simulink model "gtm_design"  (R2021b)
settings: Solver=VariableStepAuto  StartTime=0.0  StopTime=10.0  MinStep=0.00999  RelTol=1e-3
StopFcn:
  | MWSout=grabmws(bdroot);
  | MWSout.lastrun=datestr(now);
values from neighbouring files (symbols this model uses):
  knots2fps = 1.68781    [setup.m]
  s = tf('s')    [setup.m]
undefined symbols (not defined in the file or in its folder): Aero, aftfuel, aftfuel_pos, AILL, AILLC, AILR, AILRC, alpha_deg, alt0, altitude_ft, Ax_g, Ay_g, Az_g, b, beta_deg, bias, BRAKEC, Cbar, cg_pos0, cg_shift_gear, ControlMode, DamageCase, DamageModels, DamageOnsetTime, deltc, Earth, ELLIB, ELLIBC, ELLOB, ELLOBC, ELRIB, ELRIBC, ELROB, ELROBC, engl_ang, engl_pos, engr_ang, engr_pos, etas0, etas1, etasc_feedthrough, FLAPLC, FLAPLIB, FLAPLOB, FLAPRC, FLAPRIB, FLAPROB, FlightMode, FuelUsed_Init, fwdfuel, fwdfuel_pos, GEAR, GEARC, Inertia0, Inertia_shift_gear, Ixx_model, Iyy_model, Izz_model, KTAS, LandingGear ... (+66)
libraries: simulink_extras x98, LPVBlockLibrary x54, simulink_need_slupdate x30, aerolibconvert2 x27, simulink x7, aerolibtransform2 x6, uavalgslib x4, UserContent_lib x2, robotcorelib x1, uavutilslib x1
(part 7 of 9)

== system gtm_design/Guidance/Autopilot Trajectory Tracking/Orbit Following/Pose ==
  Feedback : Inport
  Bus Creator : BusCreator  Inputs=8
  Bus Selector : BusSelector  OutputSignals=AirData.KTAS
  Bus Selector1 : BusSelector  OutputSignals=MIDG.NAV_Vu_mps,MIDG.NAV_Vn_mps,MIDG.NAV_Ve_mps
  Bus Selector2 : BusSelector  OutputSignals=MIDG.NAV_Ve_mps,MIDG.NAV_Vn_mps
  Bus Selector3 : BusSelector  OutputSignals=MIDG.NAV_latitude_deg,MIDG.NAV_longitude_deg,MIDG.NAV_altitude_m
  Bus Selector4 : BusSelector  OutputSignals=MIDG.phi_deg,MAG3.p_deg
  Bus Selector6 : BusSelector  OutputSignals=North,East,Height,HeadingAngle  OutputAsBus=on
  Bus to Vector : BusToVector
  Bus to Vector1 : BusToVector
  Bus to Vector2 : BusToVector
  Constant1 : Constant  Value=[37.827926944;-75.494061666]
  Constant2 : Constant  Value=0
  Constant3 : Constant  Value=0
  Degrees to Radians{,1..3} (4 alike) : simulink_extras/Transformations/Degrees to Radians
  Demux1 : Demux  Outputs=3
      settings: DisplayOption=none
  Gain : Gain  Gain=-1
  LLA to Flat Earth : aerolibtransform2/LLA to Flat Earth  units=Metric (MKS)  ptype=Earth (WGS84)  F=1/298.257223563  R=6378137  refPosPort=on  LL0=[0 10]  psi=0
      settings: SourceProductBaseCode=AE
  Map 0_1 : Subsystem
  Mux : Mux  Inputs=2
  Mux2 : Mux  Inputs=2
  Trigonometric Function1 : Trigonometry  Operator=atan2
  Trigonometric Function3 : Trigonometry  Operator=atan2
  VecNorm : Subsystem
  Velocity Conversion : aerolibconvert2/Velocity Conversion  IU=kts  OU=m/s
  fpstoknots2 : Gain  Gain=180/pi
  Pose : Outport
  wires:
  Bus Selector2/2 -> Trigonometric Function3/2  "<NAV_Vn_mps>"
  Trigonometric Function3/1 -> Map 0_1/1(I)  "gndtrack"
  Map 0_1/1(O) -> Degrees to Radians/1  "HeadingAngle"
  Bus Selector2/1 -> Trigonometric Function3/1  "<NAV_Ve_mps>"
  Feedback/1 -> Bus Selector/1, Bus Selector4/1, Bus Selector1/1, Bus Selector2/1, Bus Selector3/1
  Mux2/1 -> LLA to Flat Earth/1
  LLA to Flat Earth/1 -> Demux1/1
  Constant1/1 -> LLA to Flat Earth/4
  Bus Selector3/2 -> Mux2/2  "<NAV_longitude_deg>"
  Bus Selector3/1 -> Mux2/1  "<NAV_latitude_deg>"
  Constant3/1 -> LLA to Flat Earth/3
  Bus Selector3/3 -> LLA to Flat Earth/2  "<NAV_altitude_m>"
  Demux1/3 -> Gain/1  "Down"
  Constant2/1 -> LLA to Flat Earth/5
  Mux/1 -> VecNorm/1(I)
  VecNorm/1(O) -> Trigonometric Function1/2
  Trigonometric Function1/1 -> fpstoknots2/1  "gamma"
  Bus Selector1/3 -> Mux/2  "<NAV_Ve_mps>"
  Bus Selector1/2 -> Mux/1  "<NAV_Vn_mps>"
  Bus Selector1/1 -> Trigonometric Function1/1  "<NAV_Vu_mps>"
  Gain/1 -> Bus Creator/3  "Height"
  Demux1/2 -> Bus Creator/2  "East"
  Demux1/1 -> Bus Creator/1  "North"
  Bus Selector/1 -> Bus to Vector/1  "<KTAS>"
  fpstoknots2/1 -> Degrees to Radians1/1  "FlightPathAngle"
  Bus Selector4/2 -> Bus to Vector2/1  "<p_deg>"
  Bus Selector4/1 -> Bus to Vector1/1  "<phi_deg>"
  Bus to Vector/1 -> Velocity Conversion/1  "KTAS"
  Bus to Vector1/1 -> Degrees to Radians2/1  "RollAngle"
  Bus to Vector2/1 -> Degrees to Radians3/1  "RollAngleRate"
  Velocity Conversion/1 -> Bus Creator/4  "AirSpeed"
  Bus Selector6/1 -> Pose/1
  Bus Creator/1 -> Bus Selector6/1
  Degrees to Radians/1 -> Bus Creator/5  "HeadingAngle"
  Degrees to Radians1/1 -> Bus Creator/6  "FlightPathAngle"
  Degrees to Radians2/1 -> Bus Creator/7  "RollAngle"
  Degrees to Radians3/1 -> Bus Creator/8  "RollAngleRate"

== system gtm_design/Guidance/Autopilot Trajectory Tracking/Waypoint Following/Pose ==
  Feedback : Inport
  Bus Creator : BusCreator  Inputs=8
  Bus Selector : BusSelector  OutputSignals=AirData.KTAS
  Bus Selector1 : BusSelector  OutputSignals=MIDG.NAV_Vu_mps,MIDG.NAV_Vn_mps,MIDG.NAV_Ve_mps
  Bus Selector2 : BusSelector  OutputSignals=MIDG.NAV_Ve_mps,MIDG.NAV_Vn_mps
  Bus Selector3 : BusSelector  OutputSignals=MIDG.NAV_latitude_deg,MIDG.NAV_longitude_deg,MIDG.NAV_altitude_m
  Bus Selector4 : BusSelector  OutputSignals=MIDG.phi_deg,MAG3.p_deg
  Bus Selector6 : BusSelector  OutputSignals=North,East,Height,HeadingAngle  OutputAsBus=on
  Bus to Vector : BusToVector
  Bus to Vector1 : BusToVector
  Bus to Vector2 : BusToVector
  Constant1 : Constant  Value=[37.827926944;-75.494061666]
  Constant2 : Constant  Value=0
  Constant3 : Constant  Value=0
  Degrees to Radians{,1..3} (4 alike) : simulink_extras/Transformations/Degrees to Radians
  Demux1 : Demux  Outputs=3
      settings: DisplayOption=none
  Gain : Gain  Gain=-1
  LLA to Flat Earth : aerolibtransform2/LLA to Flat Earth  units=Metric (MKS)  ptype=Earth (WGS84)  F=1/298.257223563  R=6378137  refPosPort=on  LL0=[0 10]  psi=0
      settings: SourceProductBaseCode=AE
  Map 0_1 : Subsystem
  Mux : Mux  Inputs=2
  Mux2 : Mux  Inputs=2
  Trigonometric Function1 : Trigonometry  Operator=atan2
  Trigonometric Function3 : Trigonometry  Operator=atan2
  VecNorm : Subsystem
  Velocity Conversion : aerolibconvert2/Velocity Conversion  IU=kts  OU=m/s
  fpstoknots2 : Gain  Gain=180/pi
  Pose : Outport
  wires:
  Degrees to Radians3/1 -> Bus Creator/8  "RollAngleRate"
  Degrees to Radians2/1 -> Bus Creator/7  "RollAngle"
  Degrees to Radians1/1 -> Bus Creator/6  "FlightPathAngle"
  Degrees to Radians/1 -> Bus Creator/5  "HeadingAngle"
  Bus Creator/1 -> Bus Selector6/1
  Bus Selector6/1 -> Pose/1
  Velocity Conversion/1 -> Bus Creator/4  "AirSpeed"
  Bus to Vector2/1 -> Degrees to Radians3/1  "RollAngleRate"
  Bus to Vector1/1 -> Degrees to Radians2/1  "RollAngle"
  Bus to Vector/1 -> Velocity Conversion/1  "KTAS"
  Bus Selector4/1 -> Bus to Vector1/1  "<phi_deg>"
  Bus Selector4/2 -> Bus to Vector2/1  "<p_deg>"
  fpstoknots2/1 -> Degrees to Radians1/1  "FlightPathAngle"
  Bus Selector/1 -> Bus to Vector/1  "<KTAS>"
  Demux1/1 -> Bus Creator/1  "North"
  Demux1/2 -> Bus Creator/2  "East"
  Gain/1 -> Bus Creator/3  "Height"
  Bus Selector1/1 -> Trigonometric Function1/1  "<NAV_Vu_mps>"
  Bus Selector1/2 -> Mux/1  "<NAV_Vn_mps>"
  Bus Selector1/3 -> Mux/2  "<NAV_Ve_mps>"
  Trigonometric Function1/1 -> fpstoknots2/1  "gamma"
  VecNorm/1(O) -> Trigonometric Function1/2
  Mux/1 -> VecNorm/1(I)
  Constant2/1 -> LLA to Flat Earth/5
  Demux1/3 -> Gain/1  "Down"
  Bus Selector3/3 -> LLA to Flat Earth/2  "<NAV_altitude_m>"
  Constant3/1 -> LLA to Flat Earth/3
  Bus Selector3/1 -> Mux2/1  "<NAV_latitude_deg>"
  Bus Selector3/2 -> Mux2/2  "<NAV_longitude_deg>"
  Constant1/1 -> LLA to Flat Earth/4
  LLA to Flat Earth/1 -> Demux1/1
  Mux2/1 -> LLA to Flat Earth/1
  Feedback/1 -> Bus Selector3/1, Bus Selector2/1, Bus Selector1/1, Bus Selector4/1, Bus Selector/1
  Bus Selector2/1 -> Trigonometric Function3/1  "<NAV_Ve_mps>"
  Map 0_1/1(O) -> Degrees to Radians/1  "HeadingAngle"
  Trigonometric Function3/1 -> Map 0_1/1(I)  "gndtrack"
  Bus Selector2/2 -> Trigonometric Function3/2  "<NAV_Vn_mps>"

== system gtm_design/Guidance/Heading Control/FlightState/Map 0_1 ==
  I : Inport
  Constant : Constant  Value=2*pi
  Constant1 : Constant  Value=0
  Gain : Gain  Gain=180/pi
  Sum : Sum  Inputs=|++
  ifnegadd2pi : Switch
  O : Outport
  wires:
  I/1 -> Sum/1, ifnegadd2pi/2
  Sum/1 -> Gain/1
  ifnegadd2pi/1 -> Sum/2
  Constant/1 -> ifnegadd2pi/3
  Constant1/1 -> ifnegadd2pi/1
  Gain/1 -> O/1

== system gtm_design/Guidance/Heading Control/FlightState/VecNorm ==
  I : Inport
  Math Function2 : Math  Operator=sqrt  SignedPower=on  SaturateOnIntegerOverflow=on
  Product : Product  RndMeth=Zero
  Sum of Elements : Sum  Inputs=+
  O : Outport
  wires:
  Sum of Elements/1 -> Math Function2/1
  Product/1 -> Sum of Elements/1
  I/1 -> Product/2, Product/1
  Math Function2/1 -> O/1

== system gtm_design/Guidance/Orbit Following/Subsystem1/Map 0_1 ==
  I : Inport
  Constant : Constant  Value=2*pi
  Constant1 : Constant  Value=0
  Gain : Gain  Gain=180/pi
  Sum : Sum  Inputs=|++
  ifnegadd2pi : Switch
  O : Outport
  wires:
  Gain/1 -> O/1
  Constant1/1 -> ifnegadd2pi/1
  Constant/1 -> ifnegadd2pi/3
  ifnegadd2pi/1 -> Sum/2
  Sum/1 -> Gain/1
  I/1 -> ifnegadd2pi/2, Sum/1

== system gtm_design/Guidance/Orbit Following/Subsystem1/VecNorm ==
  I : Inport
  Math Function2 : Math  Operator=sqrt  SignedPower=on  SaturateOnIntegerOverflow=on
  Product : Product  RndMeth=Zero
  Sum of Elements : Sum  Inputs=+
  O : Outport
  wires:
  Math Function2/1 -> O/1
  I/1 -> Product/1, Product/2
  Product/1 -> Sum of Elements/1
  Sum of Elements/1 -> Math Function2/1

== system gtm_design/Guidance/Waypoint Following/Subsystem1/Map 0_1 ==
  I : Inport
  Constant : Constant  Value=2*pi
  Constant1 : Constant  Value=0
  Gain : Gain  Gain=180/pi
  Sum : Sum  Inputs=|++
  ifnegadd2pi : Switch
  O : Outport
  wires:
  I/1 -> Sum/1, ifnegadd2pi/2
  Sum/1 -> Gain/1
  ifnegadd2pi/1 -> Sum/2
  Constant/1 -> ifnegadd2pi/3
  Constant1/1 -> ifnegadd2pi/1
  Gain/1 -> O/1

== system gtm_design/Guidance/Waypoint Following/Subsystem1/VecNorm ==
  I : Inport
  Math Function2 : Math  Operator=sqrt  SignedPower=on  SaturateOnIntegerOverflow=on
  Product : Product  RndMeth=Zero
  Sum of Elements : Sum  Inputs=+
  O : Outport
  wires:
  Sum of Elements/1 -> Math Function2/1
  Product/1 -> Sum of Elements/1
  I/1 -> Product/2, Product/1
  Math Function2/1 -> O/1

== system gtm_design/Control/Controller/Control Algorithm/Hinf Autopilot/Lateral-Directional Controller ==
  cmd_autopilot_lat : Inport
  feedback : Inport  Port=2
  Bus Selector : BusSelector  OutputSignals=bet_c_deg,phi_c_deg  OutputAsBus=on
  Bus to Vector : BusToVector
  Degrees to Radians : simulink_extras/Transformations/Degrees to Radians
  Degrees to Radians1 : simulink_extras/Transformations/Degrees to Radians
  Demux : Demux  Outputs=3
  Demux1 : Demux  Outputs=2
  Demux2 : Demux  Outputs=[1 2 1]
  Full State : Subsystem
  Linear Controller : LPVBlockLibrary/LPVBlock  sys=Klat4hinf  plist={'rho1_sas_param';'rho2_alt_param';'rho3_mor_param'}  x0=0
      settings: SourceProductName=LPVTools Blocks
  Mux : Mux  Inputs=2
  Mux1 : Mux  Inputs=2
  Mux2 : Mux  Inputs=2
  Scheduling Parameter : Subsystem
  Sum : Sum  Inputs=|+-
  Sum1 : Sum  Inputs=|+-
  Sum2 : Sum  Inputs=|++
  Sum3 : Sum  Inputs=|+-
  Trim Command : Subsystem
  Trim Input : Subsystem
  Trim State : Subsystem
  feedback1 : InportShadow  Port=2
  AILC : Outport
  RUDC : Outport  Port=2
  SPANAC : Outport  Port=3
  wires:
  Demux/1 -> AILC/1
  Degrees to Radians1/1 -> Mux1/2  "phi_c_rad"
  Degrees to Radians/1 -> Mux1/1  "bet_c_rad"
  feedback/1 -> Scheduling Parameter/1(feedback)
  cmd_autopilot_lat/1 -> Bus Selector/1
  Bus Selector/1 -> Bus to Vector/1  "r"
  feedback1/1 -> Full State/1(feedback)
  Full State/1(x) -> Sum1/1  "x"
  Sum1/1 -> Demux2/1  "dx"
  Demux/2 -> RUDC/1
  Demux/3 -> SPANAC/1
  Scheduling Parameter/1(rho) -> [rho]
  [rho] -> Trim Command/1(rho)
  [rho] -> Trim Input/1(rho)
  [rho] -> Trim State/1(rho)
  [rho] -> Linear Controller/2
  Sum2/1 -> Demux/1  "u"
  Trim Input/1(x_eq) -> Sum2/2
  Sum/1 -> Sum3/1  "dr"
  Mux/1 -> Linear Controller/1
  Trim State/1(x_eq) -> Sum1/2  "x_eq"
  Linear Controller/1 -> Sum2/1  "du"
  Mux1/1 -> Sum/1  "r"
  Trim Command/1(r_eq) -> Sum/2
  Bus to Vector/1 -> Demux1/1  "r"
  Demux1/1 -> Degrees to Radians/1  "bet_c_deg"
  Demux1/2 -> Degrees to Radians1/1  "phi_c_deg"
  Mux2/1 -> Sum3/2
  Sum3/1 -> Mux/1  "dx"
  Demux2/2 -> Mux/2
  Demux2/1 -> Mux2/1
  Demux2/3 -> Mux2/2

== system gtm_design/Control/Controller/Control Algorithm/Hinf Autopilot/Longitudinal Controller ==
  cmd_autopilot_lon : Inport
  feedback : Inport  Port=2
  Bus Selector : BusSelector  OutputSignals=tas_c_knot,alt_c_ft  OutputAsBus=on
  Bus to Vector : BusToVector
  Demux : Demux  Outputs=2
  Demux1 : Demux  Outputs=2
  Demux2 : Demux  Outputs=[1 3 1]
  Full State : Subsystem
  Linear Controller : LPVBlockLibrary/LPVBlock  sys=Klon5hinf  plist={'rho1_sas_param';'rho2_alt_param';'rho3_mor_param'}  x0=0
      settings: SourceProductName=LPVTools Blocks
  Mux : Mux  Inputs=2
  Mux1 : Mux  Inputs=2
  Mux2 : Mux  Inputs=2
  Scheduling Parameter : Subsystem
  Sum : Sum  Inputs=|+-
  Sum1 : Sum  Inputs=|+-
  Sum2 : Sum  Inputs=|++
  Sum3 : Sum  Inputs=|+-
  Trim Command : Subsystem
  Trim Input : Subsystem
  Trim State : Subsystem
  feedback1 : InportShadow  Port=2
  knotstofps : Gain  Gain=knots2fps
  THROTC : Outport
  ELLC : Outport  Port=2
  wires:
  Demux2/3 -> Mux2/2
  Demux2/1 -> Mux2/1
  Demux2/2 -> Mux/2
  Sum3/1 -> Mux/1  "dx"
  Mux2/1 -> Sum3/2
  knotstofps/1 -> Mux1/1  "tas_trim_fps"
  Demux1/1 -> knotstofps/1
  Bus to Vector/1 -> Demux1/1  "r"
  Trim Command/1(r_eq) -> Sum/2
  Mux1/1 -> Sum/1  "r"
  Linear Controller/1 -> Sum2/1  "du"
  Trim State/1(x_eq) -> Sum1/2  "x_eq"
  Mux/1 -> Linear Controller/1
  Sum/1 -> Sum3/1  "dr"
  Trim Input/1(u_eq) -> Sum2/2
  Sum2/1 -> Demux/1  "u"
  [rho] -> Linear Controller/2
  [rho] -> Trim State/1(rho)
  [rho] -> Trim Input/1(rho)
  [rho] -> Trim Command/1(rho)
  Scheduling Parameter/1(rho) -> [rho]
  Demux/2 -> ELLC/1
  Demux/1 -> THROTC/1
  Sum1/1 -> Demux2/1  "dx"
  Full State/1(x) -> Sum1/1  "x"
  feedback1/1 -> Full State/1(feedback)
  Bus Selector/1 -> Bus to Vector/1  "r"
  cmd_autopilot_lon/1 -> Bus Selector/1
  feedback/1 -> Scheduling Parameter/1(feedback)
  Demux1/2 -> Mux1/2

== system gtm_design/Control/Controller/Control Algorithm/Hinf CAS/Lateral-Directional Controller ==
  cmd_cas_lat : Inport
  feedback : Inport  Port=2
  Bus Selector : BusSelector  OutputSignals=bet_c_deg,p_c_deg  OutputAsBus=on
  Bus to Vector : BusToVector
  Degrees to Radians : simulink_extras/Transformations/Degrees to Radians
  Degrees to Radians1 : simulink_extras/Transformations/Degrees to Radians
  Demux : Demux  Outputs=3
  Demux1 : Demux  Outputs=2
  Demux2 : Demux  Outputs=[2 1]
  Full State : Subsystem
  Linear Controller : LPVBlockLibrary/LPVBlock  sys=Klat3hinf  plist={'rho1_sas_param';'rho2_alt_param';'rho3_mor_param'}  x0=0
      settings: SourceProductName=LPVTools Blocks
  Mux : Mux  Inputs=2
  Mux1 : Mux  Inputs=2
  Scheduling Parameter : Subsystem
  Sum : Sum  Inputs=|+-
  Sum1 : Sum  Inputs=|+-
  Sum2 : Sum  Inputs=|++
  Sum3 : Sum  Inputs=|+-
  Trim Command : Subsystem
  Trim Input : Subsystem
  Trim State : Subsystem
  feedback1 : InportShadow  Port=2
  AILC : Outport
  RUDC : Outport  Port=2
  SPANAC : Outport  Port=3
  wires:
  Sum3/1 -> Mux/1  "dx"
  Demux1/2 -> Degrees to Radians1/1  "p_c_deg"
  Demux1/1 -> Degrees to Radians/1  "bet_c_deg"
  Bus to Vector/1 -> Demux1/1  "r"
  Trim Command/1(r_eq) -> Sum/2
  Mux1/1 -> Sum/1  "r"
  Linear Controller/1 -> Sum2/1  "du"
  Trim State/1(x_eq) -> Sum1/2  "x_eq"
  Mux/1 -> Linear Controller/1
  Sum/1 -> Sum3/1  "dr"
  Trim Input/1(x_eq) -> Sum2/2
  Sum2/1 -> Demux/1  "u"
  [rho] -> Linear Controller/2
  [rho] -> Trim State/1(rho)
  [rho] -> Trim Input/1(rho)
  [rho] -> Trim Command/1(rho)
  Scheduling Parameter/1(rho) -> [rho]
  Demux/3 -> SPANAC/1
  Demux/2 -> RUDC/1
  Sum1/1 -> Demux2/1  "dx"
  Full State/1(x) -> Sum1/1  "x"
  feedback1/1 -> Full State/1(feedback)
  Bus Selector/1 -> Bus to Vector/1  "r"
  cmd_cas_lat/1 -> Bus Selector/1
  feedback/1 -> Scheduling Parameter/1(feedback)
  Degrees to Radians/1 -> Mux1/1  "bet_c_rad"
  Degrees to Radians1/1 -> Mux1/2  "p_c_rad"
  Demux/1 -> AILC/1
  Demux2/2 -> Mux/2
  Demux2/1 -> Sum3/2

== system gtm_design/Control/Controller/Control Algorithm/Hinf CAS/Longitudinal Controller ==
  cmd_cas_lon : Inport
  feedback : Inport  Port=2
  Bus Selector : BusSelector  OutputSignals=an_c_g  OutputAsBus=on
  Bus to Vector : BusToVector
  Constant : Constant  Value=deltc
  Demux2 : Demux  Outputs=[2 1]
  Full State : Subsystem
  Gain : Gain  Gain=-1
  Linear Controller : LPVBlockLibrary/LPVBlock  sys=Klon2hinf  plist={'rho1_sas_param';'rho2_alt_param';'rho3_mor_param'}  x0=0
      settings: SourceProductName=LPVTools Blocks
  Mux : Mux  Inputs=2
  Scheduling Parameter : Subsystem
  Sum : Sum  Inputs=|+-
  Sum1 : Sum  Inputs=|+-
  Sum2 : Sum  Inputs=|++
  Sum3 : Sum  Inputs=|+-
  Trim Command : Subsystem
  Trim Input : Subsystem
  Trim State : Subsystem
  feedback1 : InportShadow  Port=2
  knotstofps : Gain  Gain=32.174
  THROTC : Outport
  ELLC : Outport  Port=2
  wires:
  feedback/1 -> Scheduling Parameter/1(feedback)
  cmd_cas_lon/1 -> Bus Selector/1
  Bus Selector/1 -> Bus to Vector/1  "r"
  feedback1/1 -> Full State/1(feedback)
  Full State/1(y) -> Sum1/1  "y"
  Sum1/1 -> Demux2/1  "dy"
  Constant/1 -> THROTC/1
  Scheduling Parameter/1(rho) -> [rho]
  [rho] -> Trim Command/1(rho)
  [rho] -> Trim Input/1(rho)
  [rho] -> Trim State/1(rho)
  [rho] -> Linear Controller/2
  Sum2/1 -> ELLC/1  "u"
  Trim Input/1(u_eq) -> Sum2/2
  Sum/1 -> Sum3/1  "dr"
  Mux/1 -> Linear Controller/1
  Trim State/1(x_eq) -> Sum1/2  "x_eq"
  Linear Controller/1 -> Sum2/1  "du"
  knotstofps/1 -> Sum/1  "r"
  Trim Command/1(r_eq) -> Sum/2  "r_eq"
  Bus to Vector/1 -> knotstofps/1  "an_c_g"
  Sum3/1 -> Mux/1  "dx"
  Demux2/2 -> Gain/1
  Demux2/1 -> Mux/2
  Gain/1 -> Sum3/2

== system gtm_design/Control/Controller/Control Algorithm/LPV Autopilot/Lateral-Directional Controller ==
  cmd_autopilot_lat : Inport
  feedback : Inport  Port=2
  Bus Selector : BusSelector  OutputSignals=bet_c_deg,phi_c_deg  OutputAsBus=on
  Bus to Vector : BusToVector
  Degrees to Radians : simulink_extras/Transformations/Degrees to Radians
  Degrees to Radians1 : simulink_extras/Transformations/Degrees to Radians
  Demux : Demux  Outputs=3
  Demux1 : Demux  Outputs=2
  Demux2 : Demux  Outputs=[1 2 1]
  Full State : Subsystem
  Linear Controller : LPVBlockLibrary/LPVBlock  sys=Klat4lpvu  plist={'rho1_sas_param';'rho2_alt_param';'rho3_mor_param'}  x0=0
      settings: SourceProductName=LPVTools Blocks
  Mux : Mux  Inputs=2
  Mux1 : Mux  Inputs=2
  Mux2 : Mux  Inputs=2
  Scheduling Parameter : Subsystem
  Sum : Sum  Inputs=|+-
  Sum1 : Sum  Inputs=|+-
  Sum2 : Sum  Inputs=|++
  Sum3 : Sum  Inputs=|+-
  Trim Command : Subsystem
  Trim Input : Subsystem
  Trim State : Subsystem
  feedback1 : InportShadow  Port=2
  AILC : Outport
  RUDC : Outport  Port=2
  SPANAC : Outport  Port=3
  wires:
  Demux2/3 -> Mux2/2
  Demux2/1 -> Mux2/1
  Demux2/2 -> Mux/2
  Sum3/1 -> Mux/1  "dx"
  Mux2/1 -> Sum3/2
  Demux1/2 -> Degrees to Radians1/1  "phi_c_deg"
  Demux1/1 -> Degrees to Radians/1  "bet_c_deg"
  Bus to Vector/1 -> Demux1/1  "r"
  Trim Command/1(r_eq) -> Sum/2
  Mux1/1 -> Sum/1  "r"
  Linear Controller/1 -> Sum2/1  "du"
  Trim State/1(x_eq) -> Sum1/2  "x_eq"
  Mux/1 -> Linear Controller/1
  Sum/1 -> Sum3/1  "dr"
  Trim Input/1(x_eq) -> Sum2/2
  Sum2/1 -> Demux/1  "u"
  [rho] -> Linear Controller/2
  [rho] -> Trim State/1(rho)
  [rho] -> Trim Input/1(rho)
  [rho] -> Trim Command/1(rho)
  Scheduling Parameter/1(rho) -> [rho]
  Demux/3 -> SPANAC/1
  Demux/2 -> RUDC/1
  Sum1/1 -> Demux2/1  "dx"
  Full State/1(x) -> Sum1/1  "x"
  feedback1/1 -> Full State/1(feedback)
  Bus Selector/1 -> Bus to Vector/1  "r"
  cmd_autopilot_lat/1 -> Bus Selector/1
  feedback/1 -> Scheduling Parameter/1(feedback)
  Degrees to Radians/1 -> Mux1/1  "bet_c_rad"
  Degrees to Radians1/1 -> Mux1/2  "phi_c_rad"
  Demux/1 -> AILC/1

== system gtm_design/Control/Controller/Control Algorithm/LPV Autopilot/Longitudinal Controller ==
  cmd_autopilot_lon : Inport
  feedback : Inport  Port=2
  Bus Selector : BusSelector  OutputSignals=tas_c_knot,alt_c_ft  OutputAsBus=on
  Bus to Vector : BusToVector
  Demux : Demux  Outputs=2
  Demux1 : Demux  Outputs=2
  Demux2 : Demux  Outputs=[1 3 1]
  Full State : Subsystem
  Linear Controller : LPVBlockLibrary/LPVBlock  sys=Klon5lpvu  plist={'rho1_sas_param';'rho2_alt_param';'rho3_mor_param'}  x0=0
      settings: SourceProductName=LPVTools Blocks
  Mux : Mux  Inputs=2
  Mux1 : Mux  Inputs=2
  Mux2 : Mux  Inputs=2
  Scheduling Parameter : Subsystem
  Sum : Sum  Inputs=|+-
  Sum1 : Sum  Inputs=|+-
  Sum2 : Sum  Inputs=|++
  Sum3 : Sum  Inputs=|+-
  Trim Command : Subsystem
  Trim Input : Subsystem
  Trim State : Subsystem
  feedback1 : InportShadow  Port=2
  knotstofps : Gain  Gain=knots2fps
  THROTC : Outport
  ELLC : Outport  Port=2
  wires:
  feedback/1 -> Scheduling Parameter/1(feedback)
  cmd_autopilot_lon/1 -> Bus Selector/1
  Bus Selector/1 -> Bus to Vector/1  "r"
  feedback1/1 -> Full State/1(feedback)
  Full State/1(x) -> Sum1/1  "x"
  Sum1/1 -> Demux2/1  "dx"
  Demux/1 -> THROTC/1
  Demux/2 -> ELLC/1
  Scheduling Parameter/1(rho) -> [rho]
  [rho] -> Trim Command/1(rho)
  [rho] -> Trim Input/1(rho)
  [rho] -> Trim State/1(rho)
  [rho] -> Linear Controller/2
  Sum2/1 -> Demux/1  "u"
  Trim Input/1(u_eq) -> Sum2/2
  Sum/1 -> Sum3/1  "dr"
  Mux/1 -> Linear Controller/1
  Trim State/1(x_eq) -> Sum1/2  "x_eq"
  Linear Controller/1 -> Sum2/1  "du"
  Mux1/1 -> Sum/1  "r"
  Trim Command/1(r_eq) -> Sum/2
  Bus to Vector/1 -> Demux1/1  "r"
  Demux1/1 -> knotstofps/1
  knotstofps/1 -> Mux1/1  "tas_trim_fps"
  Mux2/1 -> Sum3/2
  Sum3/1 -> Mux/1  "dx"
  Demux2/2 -> Mux/2
  Demux2/1 -> Mux2/1
  Demux2/3 -> Mux2/2
  Demux1/2 -> Mux1/2

== system gtm_design/Control/Controller/Control Algorithm/LPV CAS/Lateral-Directional Controller ==
  cmd_cas_lat : Inport
  feedback : Inport  Port=2
  Bus Selector : BusSelector  OutputSignals=bet_c_deg,p_c_deg  OutputAsBus=on
  Bus to Vector : BusToVector
  Degrees to Radians : simulink_extras/Transformations/Degrees to Radians
  Degrees to Radians1 : simulink_extras/Transformations/Degrees to Radians
  Demux : Demux  Outputs=3
  Demux1 : Demux  Outputs=2
  Demux2 : Demux  Outputs=[2 1]
  Full State : Subsystem
  Linear Controller : LPVBlockLibrary/LPVBlock  sys=Klat3lpvu  plist={'rho1_sas_param';'rho2_alt_param';'rho3_mor_param'}  x0=0
      settings: SourceProductName=LPVTools Blocks
  Mux : Mux  Inputs=2
  Mux1 : Mux  Inputs=2
  Scheduling Parameter : Subsystem
  Sum : Sum  Inputs=|+-
  Sum1 : Sum  Inputs=|+-
  Sum2 : Sum  Inputs=|++
  Sum3 : Sum  Inputs=|+-
  Trim Command : Subsystem
  Trim Input : Subsystem
  Trim State : Subsystem
  feedback1 : InportShadow  Port=2
  AILC : Outport
  RUDC : Outport  Port=2
  SPANAC : Outport  Port=3
  wires:
  Demux/1 -> AILC/1
  Degrees to Radians1/1 -> Mux1/2  "p_c_rad"
  Degrees to Radians/1 -> Mux1/1  "bet_c_rad"
  feedback/1 -> Scheduling Parameter/1(feedback)
  cmd_cas_lat/1 -> Bus Selector/1
  Bus Selector/1 -> Bus to Vector/1  "r"
  feedback1/1 -> Full State/1(feedback)
  Full State/1(x) -> Sum1/1  "x"
  Sum1/1 -> Demux2/1  "dx"
  Demux/2 -> RUDC/1
  Demux/3 -> SPANAC/1
  Scheduling Parameter/1(rho) -> [rho]
  [rho] -> Trim Command/1(rho)
  [rho] -> Trim Input/1(rho)
  [rho] -> Trim State/1(rho)
  [rho] -> Linear Controller/2
  Sum2/1 -> Demux/1  "u"
  Trim Input/1(x_eq) -> Sum2/2
  Sum/1 -> Sum3/1  "dr"
  Mux/1 -> Linear Controller/1
  Trim State/1(x_eq) -> Sum1/2  "x_eq"
  Linear Controller/1 -> Sum2/1  "du"
  Mux1/1 -> Sum/1  "r"
  Trim Command/1(r_eq) -> Sum/2
  Bus to Vector/1 -> Demux1/1  "r"
  Demux1/1 -> Degrees to Radians/1  "bet_c_deg"
  Demux1/2 -> Degrees to Radians1/1  "p_c_deg"
  Sum3/1 -> Mux/1  "dx"
  Demux2/2 -> Mux/2
  Demux2/1 -> Sum3/2

== system gtm_design/Control/Controller/Control Algorithm/LPV CAS/Longitudinal Controller ==
  cmd_cas_lon : Inport
  feedback : Inport  Port=2
  Bus Selector : BusSelector  OutputSignals=an_c_g  OutputAsBus=on
  Bus to Vector : BusToVector
  Constant : Constant  Value=deltc
  Demux2 : Demux  Outputs=[2 1]
  Full State : Subsystem
  Gain : Gain  Gain=-1
  Linear Controller : LPVBlockLibrary/LPVBlock  sys=Klon2lpvu  plist={'rho1_sas_param';'rho2_alt_param';'rho3_mor_param'}  x0=0
      settings: SourceProductName=LPVTools Blocks
  Mux : Mux  Inputs=2
  Scheduling Parameter : Subsystem
  Sum : Sum  Inputs=|+-
  Sum1 : Sum  Inputs=|+-
  Sum2 : Sum  Inputs=|++
  Sum3 : Sum  Inputs=|+-
  Trim Command : Subsystem
  Trim Input : Subsystem
  Trim State : Subsystem
  feedback1 : InportShadow  Port=2
  knotstofps : Gain  Gain=32.174
  THROTC : Outport
  ELLC : Outport  Port=2
  wires:
  Gain/1 -> Sum3/2
  Demux2/1 -> Mux/2
  Demux2/2 -> Gain/1
  Sum3/1 -> Mux/1  "dx"
  Bus to Vector/1 -> knotstofps/1  "an_c_g"
  Trim Command/1(r_eq) -> Sum/2  "r_eq"
  knotstofps/1 -> Sum/1  "r"
  Linear Controller/1 -> Sum2/1  "du"
  Trim State/1(x_eq) -> Sum1/2  "x_eq"
  Mux/1 -> Linear Controller/1
  Sum/1 -> Sum3/1  "dr"
  Trim Input/1(u_eq) -> Sum2/2
  Sum2/1 -> ELLC/1  "u"
  [rho] -> Linear Controller/2
  [rho] -> Trim State/1(rho)
  [rho] -> Trim Input/1(rho)
  [rho] -> Trim Command/1(rho)
  Scheduling Parameter/1(rho) -> [rho]
  Constant/1 -> THROTC/1
  Sum1/1 -> Demux2/1  "dy"
  Full State/1(y) -> Sum1/1  "y"
  feedback1/1 -> Full State/1(feedback)
  Bus Selector/1 -> Bus to Vector/1  "r"
  cmd_cas_lon/1 -> Bus Selector/1
  feedback/1 -> Scheduling Parameter/1(feedback)

== system gtm_design/GTM_T2/A//C parameters/Inertia//Mass//CG Shift/FuelBurnEffects/Polyval ==
  In1 : Inport
  Embedded MATLAB Function : MATLAB Function  TreatAsAtomicUnit=on
  Out1 : Outport
  wires:
  In1/1 -> Embedded MATLAB Function/1(u)
  Embedded MATLAB Function/1(y) -> Out1/1

== system gtm_design/GTM_T2/A//C parameters/Inertia//Mass//CG Shift/FuelBurnEffects/Polyval1 ==
  In1 : Inport
  Embedded MATLAB Function : MATLAB Function  TreatAsAtomicUnit=on
  Out1 : Outport
  wires:
  In1/1 -> Embedded MATLAB Function/1(u)
  Embedded MATLAB Function/1(y) -> Out1/1

== system gtm_design/GTM_T2/A//C parameters/Inertia//Mass//CG Shift/FuelBurnEffects/Polyval2 ==
  In1 : Inport
  Embedded MATLAB Function : MATLAB Function  TreatAsAtomicUnit=on
  Out1 : Outport
  wires:
  In1/1 -> Embedded MATLAB Function/1(u)
  Embedded MATLAB Function/1(y) -> Out1/1

== system gtm_design/GTM_T2/Actuators/InputModification for Trimming/LinearizeMode:DetlasOnTrimBias/Surface Allocation For Linearizing ==
  I : Inport
  BiasSurfs : Subsystem
  Demux : Demux  Outputs=19
  Gain1 : Gain  Gain=-1
  Ground1 : Ground
  Ground2 : Ground
  Ground5 : Ground
  Mux : Mux  Inputs=22
  O : Outport
  wires:
  BiasSurfs/1(cmds) -> O/1
  I/1 -> Demux/1
  Mux/1 -> BiasSurfs/1(dCmd)
  Ground1/1 -> Mux/18  "dgear"
  Ground2/1 -> Mux/19  "dbrake"
  Ground5/1 -> Mux/22  "dSteer"
  Demux/1 -> Mux/1  "dElevatorLOB"
  Demux/2 -> Mux/2  "dElevatorLIB"
  Demux/3 -> Mux/3  "dElevatorROB"
  Demux/4 -> Mux/4  "dElevatorRIB"
  Demux/5 -> Gain1/1  "dAileronL"
  Demux/6 -> Mux/6  "dAileronR"
  Demux/7 -> Mux/7  "dRudderUpper"
  Demux/8 -> Mux/8  "dRudderLower"
  Demux/9 -> Mux/9  "dSpoilerLIB"
  Demux/10 -> Mux/10  "dSpoilerLOB"
  Demux/11 -> Mux/11  "dSpoilerRIB"
  Demux/12 -> Mux/12  "dSpoilerROB"
  Demux/13 -> Mux/13  "dFlapLIB"
  Demux/14 -> Mux/14  "dFlapLOB"
  Demux/15 -> Mux/15  "dFlapRIB"
  Demux/16 -> Mux/16  "dFlapROB"
  Demux/17 -> Mux/17  "dStabilizer"
  Demux/18 -> Mux/20  "dThrottleL"
  Demux/19 -> Mux/21  "dThrottleR"
  Gain1/1 -> Mux/5  "dAileronL"

== system gtm_design/GTM_T2/Actuators/InputModification for Trimming/TrimMode: DriveFromTopLevel/Force Consistent Sample Time on Bus ==
  In1 : Inport
  Bus to Vector : BusToVector
  Map4 : Gain
  Out1 : Outport
  wires:
  In1/1 -> Bus to Vector/1
  Map4/1 -> Out1/1
  Bus to Vector/1 -> Map4/1

== system gtm_design/GTM_T2/Actuators/InputModification for Trimming/TrimMode: DriveFromTopLevel/InitializeBus ==
  Bus Creator : BusCreator  Inputs=22
  Constant : Constant  Value=zeros(22,1)
  Demux : Demux  Outputs=22
  O : Outport
  wires:
  Constant/1 -> Demux/1
  Demux/18 -> Bus Creator/18  "GEAR"
  Demux/19 -> Bus Creator/19  "BRAKE"
  Demux/20 -> Bus Creator/20  "THROTL"
  Demux/21 -> Bus Creator/21  "THROTR"
  Demux/22 -> Bus Creator/22  "STEER"
  Demux/17 -> Bus Creator/17  "STAB"
  Bus Creator/1 -> O/1
  Demux/2 -> Bus Creator/2  "ELLIB"
  Demux/3 -> Bus Creator/3  "ELROB"
  Demux/4 -> Bus Creator/4  "ELRIB"
  Demux/5 -> Bus Creator/5  "AILL"
  Demux/6 -> Bus Creator/6  "AILR"
  Demux/7 -> Bus Creator/7  "RUDU"
  Demux/8 -> Bus Creator/8  "RUDL"
  Demux/9 -> Bus Creator/9  "SPLLIB"
  Demux/10 -> Bus Creator/10  "SPLLOB"
  Demux/11 -> Bus Creator/11  "SPLRIB"
  Demux/12 -> Bus Creator/12  "SPLROB"
  Demux/13 -> Bus Creator/13  "FLAPLIB"
  Demux/14 -> Bus Creator/14  "FLAPLOB"
  Demux/15 -> Bus Creator/15  "FLAPRIB"
  Demux/16 -> Bus Creator/16  "FLAPROB"
  Demux/1 -> Bus Creator/1  "ELLOB"

== system gtm_design/GTM_T2/Actuators/InputModification for Trimming/TrimMode: DriveFromTopLevel/MapPitchSurf ==
  UseStab : Inport
  In : Inport  Port=2
  Merge : Merge
  Switch Case : SwitchCase
  UseElevatorToTrim : Subsystem  TreatAsAtomicUnit=on
  UseStabToTrim : Subsystem  TreatAsAtomicUnit=on
  Out : Outport
  wires:
  UseElevatorToTrim/1(Out) -> Merge/1
  UseStabToTrim/1(Out1) -> Merge/2
  In/1 -> UseStabToTrim/1(In), UseElevatorToTrim/1(In)
  Merge/1 -> Out/1
  Switch Case/2 -> UseElevatorToTrim/Action
  UseStab/1 -> Switch Case/1
  Switch Case/1 -> UseStabToTrim/Action

== system gtm_design/GTM_T2/Aero/Basic Airframe/DamageEffects/Switch Case Action Subsystem ==
  alpha : Inport
  beta : Inport  Port=2
  damage_case : Inport  Port=3
  Action Port : ActionPort  ActionPortLabel=case [ 1 2 3 4 5 6 ]:
  AlphaLookup : PreLookup  BreakpointsData=Aero.dC6_damage.bas.alpha  BeginIndexSearchUsingPreviousIndexResult=on  ExtrapMethod=Linear
  BetaLookup : PreLookup  BreakpointsData=Aero.dC6_damage.bas.beta  ExtrapMethod=Linear
  Constant : Constant  Value=uint32(1)
  Constant4 : Constant  Value=[0:5]  OutDataTypeStr=uint32
  Interpolation Using Prelookup : Interpolation_n-D  NumberOfTableDimensions=4  Table=Aero.dC6_damage.bas.data  ExtrapMethod=Clip  NumSelectionDims=2
      settings: InputPortMap=u0,u1,u2,u3,u4,u5
  Subtract : Sum  Inputs=+-
  dC6_dam : Outport  InitialOutput=zeros(6,1)
  wires:
  Constant/1 -> Subtract/2
  Subtract/1 -> Interpolation Using Prelookup/5
  damage_case/1 -> Subtract/1
  BetaLookup/2 -> Interpolation Using Prelookup/4
  BetaLookup/1 -> Interpolation Using Prelookup/3
  AlphaLookup/2 -> Interpolation Using Prelookup/2
  AlphaLookup/1 -> Interpolation Using Prelookup/1
  Interpolation Using Prelookup/1 -> dC6_dam/1
  beta/1 -> BetaLookup/1
  alpha/1 -> AlphaLookup/1
  Constant4/1 -> Interpolation Using Prelookup/6

== system gtm_design/GTM_T2/Aero/Basic Airframe/DamageEffects/Switch Case Action Subsystem2 ==
  Action Port : ActionPort  ActionPortLabel=default:
  Constant4 : Constant  Value=zeros(6,1)  OutDataTypeStr=double
  Zeros : Outport  InitialOutput=zeros(6,1)
  wires:
  Constant4/1 -> Zeros/1

== system gtm_design/GTM_T2/Aero/Control Surfaces/Elevator//Stab1/RollYaw Coupling LIB ==
  I : Inport
  Gain : Gain  Gain=Kc  Multiplication=Matrix(K*u)
  O : Outport
  wires:
  Gain/1 -> O/1
  I/1 -> Gain/1

== system gtm_design/GTM_T2/Aero/Control Surfaces/Elevator//Stab1/RollYaw Coupling LOB ==
  I : Inport
  Gain : Gain  Gain=Kc  Multiplication=Matrix(K*u)
  O : Outport
  wires:
  Gain/1 -> O/1
  I/1 -> Gain/1

== system gtm_design/GTM_T2/Aero/Control Surfaces/Elevator//Stab1/RollYaw Coupling RIB ==
  I : Inport
  Gain : Gain  Gain=Kc  Multiplication=Matrix(K*u)
  O : Outport
  wires:
  Gain/1 -> O/1
  I/1 -> Gain/1

== system gtm_design/GTM_T2/Aero/Control Surfaces/Elevator//Stab1/RollYaw Coupling ROB ==
  I : Inport
  Gain : Gain  Gain=Kc  Multiplication=Matrix(K*u)
  O : Outport
  wires:
  Gain/1 -> O/1
  I/1 -> Gain/1

== system gtm_design/GTM_T2/Aero/Control Surfaces/Elevator//Stab1/Stab//Elev Table ==
  alpha_k : Inport
  alpha_f : Inport  Port=2
  beta_k : Inport  Port=3
  beta_f : Inport  Port=4
  stab_k : Inport  Port=5
  stab_f : Inport  Port=6
  elev : Inport  Port=7
  Assignment to Longitudinal : Assignment  IndexMode=Zero-based  IndexOptions=Index vector (dialog)  Indices=[0 2 4]  OutputSizes=[1 1]
  Constant : Constant  Value=zeros(6,1)
  Constant2 : Constant  Value=[0:2]  OutDataTypeStr=uint32
  Interpolation Using Prelookup : Interpolation_n-D  NumberOfTableDimensions=5  Table=Aero.dC3_ele.data  NumSelectionDims=1
      settings: InputPortMap=u0,u1,u2,u3,u4,u5,u6,u7,u8
  Prelookup4 : PreLookup  BreakpointsData=Aero.dC3_ele.elev  IndexSearchMethod=Linear search  BeginIndexSearchUsingPreviousIndexResult=on  ExtrapMethod=Linear
  dC6 : Outport
  wires:
  Constant2/1 -> Interpolation Using Prelookup/9
  Prelookup4/2 -> Interpolation Using Prelookup/8
  Prelookup4/1 -> Interpolation Using Prelookup/7
  stab_f/1 -> Interpolation Using Prelookup/6
  beta_f/1 -> Interpolation Using Prelookup/4
  alpha_f/1 -> Interpolation Using Prelookup/2
  alpha_k/1 -> Interpolation Using Prelookup/1
  beta_k/1 -> Interpolation Using Prelookup/3
  stab_k/1 -> Interpolation Using Prelookup/5
  elev/1 -> Prelookup4/1
  Constant/1 -> Assignment to Longitudinal/1
  Interpolation Using Prelookup/1 -> Assignment to Longitudinal/2
  Assignment to Longitudinal/1 -> dC6/1

== system gtm_design/GTM_T2/Aero/Control Surfaces/Elevator//Stab1/Stab//Elev Table0 ==
  alpha_k : Inport
  alpha_f : Inport  Port=2
  beta_k : Inport  Port=3
  beta_f : Inport  Port=4
  stab_k : Inport  Port=5
  stab_f : Inport  Port=6
  elev : Inport  Port=7
  Assignment to Longitudinal : Assignment  IndexMode=Zero-based  IndexOptions=Index vector (dialog)  Indices=[0 2 4]  OutputSizes=[1 1]
  Constant : Constant  Value=zeros(6,1)
  Constant2 : Constant  Value=[0:2]  OutDataTypeStr=uint32
  Interpolation Using Prelookup : Interpolation_n-D  NumberOfTableDimensions=5  Table=Aero.dC3_ele.data  NumSelectionDims=1
      settings: InputPortMap=u0,u1,u2,u3,u4,u5,u6,u7,u8
  Prelookup4 : PreLookup  BreakpointsData=Aero.dC3_ele.elev  IndexSearchMethod=Linear search  BeginIndexSearchUsingPreviousIndexResult=on  ExtrapMethod=Linear
  dC6 : Outport
  wires:
  Constant2/1 -> Interpolation Using Prelookup/9
  Prelookup4/2 -> Interpolation Using Prelookup/8
  Prelookup4/1 -> Interpolation Using Prelookup/7
  stab_f/1 -> Interpolation Using Prelookup/6
  beta_f/1 -> Interpolation Using Prelookup/4
  alpha_f/1 -> Interpolation Using Prelookup/2
  alpha_k/1 -> Interpolation Using Prelookup/1
  beta_k/1 -> Interpolation Using Prelookup/3
  stab_k/1 -> Interpolation Using Prelookup/5
  elev/1 -> Prelookup4/1
  Constant/1 -> Assignment to Longitudinal/1
  Interpolation Using Prelookup/1 -> Assignment to Longitudinal/2
  Assignment to Longitudinal/1 -> dC6/1

== system gtm_design/GTM_T2/Aero/Control Surfaces/Elevator//Stab1/Stab//Elev Table1 ==
  alpha_k : Inport
  alpha_f : Inport  Port=2
  beta_k : Inport  Port=3
  beta_f : Inport  Port=4
  stab_k : Inport  Port=5
  stab_f : Inport  Port=6
  elev : Inport  Port=7
  Assignment to Longitudinal : Assignment  IndexMode=Zero-based  IndexOptions=Index vector (dialog)  Indices=[0 2 4]  OutputSizes=[1 1]
  Constant : Constant  Value=zeros(6,1)
  Constant2 : Constant  Value=[0:2]  OutDataTypeStr=uint32
  Interpolation Using Prelookup : Interpolation_n-D  NumberOfTableDimensions=5  Table=Aero.dC3_ele.data  NumSelectionDims=1
      settings: InputPortMap=u0,u1,u2,u3,u4,u5,u6,u7,u8
  Prelookup4 : PreLookup  BreakpointsData=Aero.dC3_ele.elev  IndexSearchMethod=Linear search  BeginIndexSearchUsingPreviousIndexResult=on  ExtrapMethod=Linear
  dC6 : Outport
  wires:
  Constant2/1 -> Interpolation Using Prelookup/9
  Prelookup4/2 -> Interpolation Using Prelookup/8
  Prelookup4/1 -> Interpolation Using Prelookup/7
  stab_f/1 -> Interpolation Using Prelookup/6
  beta_f/1 -> Interpolation Using Prelookup/4
  alpha_f/1 -> Interpolation Using Prelookup/2
  alpha_k/1 -> Interpolation Using Prelookup/1
  beta_k/1 -> Interpolation Using Prelookup/3
  stab_k/1 -> Interpolation Using Prelookup/5
  elev/1 -> Prelookup4/1
  Constant/1 -> Assignment to Longitudinal/1
  Interpolation Using Prelookup/1 -> Assignment to Longitudinal/2
  Assignment to Longitudinal/1 -> dC6/1

== system gtm_design/GTM_T2/Aero/Control Surfaces/Elevator//Stab1/Stab//Elev Table2 ==
  alpha_k : Inport
  alpha_f : Inport  Port=2
  beta_k : Inport  Port=3
  beta_f : Inport  Port=4
  stab_k : Inport  Port=5
  stab_f : Inport  Port=6
  elev : Inport  Port=7
  Assignment to Longitudinal : Assignment  IndexMode=Zero-based  IndexOptions=Index vector (dialog)  Indices=[0 2 4]  OutputSizes=[1 1]
  Constant : Constant  Value=zeros(6,1)
  Constant2 : Constant  Value=[0:2]  OutDataTypeStr=uint32
  Interpolation Using Prelookup : Interpolation_n-D  NumberOfTableDimensions=5  Table=Aero.dC3_ele.data  NumSelectionDims=1
      settings: InputPortMap=u0,u1,u2,u3,u4,u5,u6,u7,u8
  Prelookup4 : PreLookup  BreakpointsData=Aero.dC3_ele.elev  IndexSearchMethod=Linear search  BeginIndexSearchUsingPreviousIndexResult=on  ExtrapMethod=Linear
  dC6 : Outport
  wires:
  Constant2/1 -> Interpolation Using Prelookup/9
  Prelookup4/2 -> Interpolation Using Prelookup/8
  Prelookup4/1 -> Interpolation Using Prelookup/7
  stab_f/1 -> Interpolation Using Prelookup/6
  beta_f/1 -> Interpolation Using Prelookup/4
  alpha_f/1 -> Interpolation Using Prelookup/2
  alpha_k/1 -> Interpolation Using Prelookup/1
  beta_k/1 -> Interpolation Using Prelookup/3
  stab_k/1 -> Interpolation Using Prelookup/5
  elev/1 -> Prelookup4/1
  Constant/1 -> Assignment to Longitudinal/1
  Interpolation Using Prelookup/1 -> Assignment to Longitudinal/2
  Assignment to Longitudinal/1 -> dC6/1

== system gtm_design/GTM_T2/Aero/Control Surfaces/Elevator//Stab1/Stab//Elev Table3 ==
  alpha_k : Inport
  alpha_f : Inport  Port=2
  beta_k : Inport  Port=3
  beta_f : Inport  Port=4
  stab_k : Inport  Port=5
  stab_f : Inport  Port=6
  elev : Inport  Port=7
  Assignment to Longitudinal : Assignment  IndexMode=Zero-based  IndexOptions=Index vector (dialog)  Indices=[0 2 4]  OutputSizes=[1 1]
  Constant : Constant  Value=zeros(6,1)
  Constant2 : Constant  Value=[0:2]  OutDataTypeStr=uint32
  Interpolation Using Prelookup : Interpolation_n-D  NumberOfTableDimensions=5  Table=Aero.dC3_ele.data  NumSelectionDims=1
      settings: InputPortMap=u0,u1,u2,u3,u4,u5,u6,u7,u8
  Prelookup4 : PreLookup  BreakpointsData=Aero.dC3_ele.elev  IndexSearchMethod=Linear search  BeginIndexSearchUsingPreviousIndexResult=on  ExtrapMethod=Linear
  dC6 : Outport
  wires:
  Constant2/1 -> Interpolation Using Prelookup/9
  Prelookup4/2 -> Interpolation Using Prelookup/8
  Prelookup4/1 -> Interpolation Using Prelookup/7
  stab_f/1 -> Interpolation Using Prelookup/6
  beta_f/1 -> Interpolation Using Prelookup/4
  alpha_f/1 -> Interpolation Using Prelookup/2
  alpha_k/1 -> Interpolation Using Prelookup/1
  beta_k/1 -> Interpolation Using Prelookup/3
  stab_k/1 -> Interpolation Using Prelookup/5
  elev/1 -> Prelookup4/1
  Constant/1 -> Assignment to Longitudinal/1
  Interpolation Using Prelookup/1 -> Assignment to Longitudinal/2
  Assignment to Longitudinal/1 -> dC6/1

== system gtm_design/GTM_T2/Aero/Control Surfaces/Flaps/Subsystem ==
  alpha : Inport
  beta : Inport  Port=2
  MORPHL : Inport  Port=3
  MORPHR : Inport  Port=4
  AlphaLookup : PreLookup  BreakpointsData=Aero.dC6_damage.bas.alpha  BeginIndexSearchUsingPreviousIndexResult=on  ExtrapMethod=Linear
  AlphaLookup1 : PreLookup  BreakpointsData=Aero.dC6_damage.bas.alpha  BeginIndexSearchUsingPreviousIndexResult=on  ExtrapMethod=Linear
  BetaLookup : PreLookup  BreakpointsData=Aero.dC6_damage.bas.beta  ExtrapMethod=Linear
  BetaLookup1 : PreLookup  BreakpointsData=Aero.dC6_damage.bas.beta  ExtrapMethod=Linear
  Constant : Constant  Value=uint32(1)
  Constant2 : Constant  Value=uint32(4)
  Constant4 : Constant  Value=[0:5]  OutDataTypeStr=uint32
  Constant5 : Constant  Value=uint32(1)
  Constant6 : Constant  Value=[0:5]  OutDataTypeStr=uint32
  Gain4 : Gain  Gain=-1/25
  Gain5 : Gain  Gain=-1
  Gain7 : Gain  Gain=-1/25
  Interpolation Using Prelookup2 : Interpolation_n-D  NumberOfTableDimensions=4  Table=Aero.dC6_damage.bas.data  ExtrapMethod=Clip  NumSelectionDims=2
      settings: InputPortMap=u0,u1,u2,u3,u4,u5
  Interpolation Using Prelookup3 : Interpolation_n-D  NumberOfTableDimensions=4  Table=Aero.dC6_damage.bas.data  ExtrapMethod=Clip  NumSelectionDims=2
      settings: InputPortMap=u0,u1,u2,u3,u4,u5
  Negate Lateral1 : Gain  Gain=[1 -1 1 -1 1 -1]
  Product : Product
  Product1 : Product
  Subtract : Sum  Inputs=+-
  Subtract1 : Sum  Inputs=+-
  LeftOutb : Outport
  RightOutb : Outport  Port=2
  wires:
  AlphaLookup/1 -> Interpolation Using Prelookup2/1
  Gain7/1 -> Product/2
  Gain5/1 -> BetaLookup1/1
  AlphaLookup1/1 -> Interpolation Using Prelookup3/1
  BetaLookup/2 -> Interpolation Using Prelookup2/4
  MORPHR/1 -> Gain4/1
  Constant4/1 -> Interpolation Using Prelookup2/6
  beta/1 -> Gain5/1, BetaLookup/1
  Subtract/1 -> Interpolation Using Prelookup2/5
  Interpolation Using Prelookup3/1 -> Negate Lateral1/1
  Product/1 -> LeftOutb/1
  Interpolation Using Prelookup2/1 -> Product/1
  Constant/1 -> Subtract/2
  AlphaLookup1/2 -> Interpolation Using Prelookup3/2
  Subtract1/1 -> Interpolation Using Prelookup3/5
  BetaLookup1/2 -> Interpolation Using Prelookup3/4
  BetaLookup/1 -> Interpolation Using Prelookup2/3
  Gain4/1 -> Product1/2
  Constant5/1 -> Subtract1/2
  Constant2/1 -> Subtract1/1, Subtract/1
  Product1/1 -> RightOutb/1
  BetaLookup1/1 -> Interpolation Using Prelookup3/3
  MORPHL/1 -> Gain7/1
  Constant6/1 -> Interpolation Using Prelookup3/6
  alpha/1 -> AlphaLookup1/1, AlphaLookup/1
  Negate Lateral1/1 -> Product1/1
  AlphaLookup/2 -> Interpolation Using Prelookup2/2

== system gtm_design/GTM_T2/Aero/Control Surfaces/Rudder/Gains ==
  dC6_in : Inport
  Product : Product  RndMeth=Zero
  gains : Constant  Value=gains
  dC6 : Outport
  wires:
  dC6_in/1 -> Product/1
  Product/1 -> dC6/1
  gains/1 -> Product/2

== system gtm_design/GTM_T2/Aero/Control Surfaces/Rudder/Gains1 ==
  dC6_in : Inport
  Product : Product  RndMeth=Zero
  gains : Constant  Value=gains
  dC6 : Outport
  wires:
  gains/1 -> Product/2
  Product/1 -> dC6/1
  dC6_in/1 -> Product/1

== system gtm_design/GTM_T2/Aero/Control Surfaces/Rudder/Lower Rudder ==
  alpha : Inport
  beta : Inport  Port=2
  rud : Inport  Port=3
  Abs : Abs
  Assignment to lateral : Assignment  IndexMode=Zero-based  IndexOptions=Index vector (dialog)  Indices=[1 3 5]  OutputSizes=[1 1]
  Constant : Constant  Value=-1
  Constant1 : Constant
  Constant2 : Constant  Value=[0:5]  OutDataTypeStr=uint32
  Constant3 : Constant  Value=ones(6,1)
  Gain : Gain  Gain=-1
  Interpolation Using Prelookup : Interpolation_n-D  NumberOfTableDimensions=4  Table=Aero.dC6_rud.data  NumSelectionDims=1
      settings: InputPortMap=u0,u1,u2,u3,u4,u5,u6
  Prelookup : PreLookup  BreakpointsData=Aero.dC6_rud.alpha  IndexSearchMethod=Linear search  BeginIndexSearchUsingPreviousIndexResult=on  ExtrapMethod=Linear
  Prelookup1 : PreLookup  BreakpointsData=Aero.dC6_rud.beta  IndexSearchMethod=Linear search  BeginIndexSearchUsingPreviousIndexResult=on  ExtrapMethod=Linear
  Prelookup2 : PreLookup  BreakpointsData=Aero.dC6_rud.rud  IndexSearchMethod=Linear search  BeginIndexSearchUsingPreviousIndexResult=on  ExtrapMethod=Linear
  Product1 : Product  RndMeth=Zero
  Product2 : Product  RndMeth=Zero
  Switch : Switch
  dC6 : Outport
  wires:
  Interpolation Using Prelookup/1 -> Product2/1
  Assignment to lateral/1 -> Product2/2
  Constant3/1 -> Assignment to lateral/1
  Switch/1 -> Assignment to lateral/2, Product1/2
  Constant1/1 -> Switch/3
  Constant/1 -> Switch/1
  Product2/1 -> dC6/1
  beta/1 -> Product1/1
  alpha/1 -> Prelookup/1
  Gain/1 -> Prelookup2/1
  Abs/1 -> Gain/1
  rud/1 -> Switch/2, Abs/1
  Product1/1 -> Prelookup1/1
  Prelookup/1 -> Interpolation Using Prelookup/1
  Prelookup/2 -> Interpolation Using Prelookup/2
  Prelookup1/1 -> Interpolation Using Prelookup/3
  Prelookup1/2 -> Interpolation Using Prelookup/4
  Prelookup2/1 -> Interpolation Using Prelookup/5
  Prelookup2/2 -> Interpolation Using Prelookup/6
  Constant2/1 -> Interpolation Using Prelookup/7

== system gtm_design/GTM_T2/Aero/Control Surfaces/Rudder/Upper Rudder ==
  alpha : Inport
  beta : Inport  Port=2
  rud : Inport  Port=3
  Abs : Abs
  Assignment to lateral : Assignment  IndexMode=Zero-based  IndexOptions=Index vector (dialog)  Indices=[1 3 5]  OutputSizes=[1 1]
  Constant : Constant  Value=-1
  Constant1 : Constant
  Constant2 : Constant  Value=[0:5]  OutDataTypeStr=uint32
  Constant3 : Constant  Value=ones(6,1)
  Gain : Gain  Gain=-1
  Interpolation Using Prelookup : Interpolation_n-D  NumberOfTableDimensions=4  Table=Aero.dC6_rud.data  NumSelectionDims=1
      settings: InputPortMap=u0,u1,u2,u3,u4,u5,u6
  Prelookup : PreLookup  BreakpointsData=Aero.dC6_rud.alpha  IndexSearchMethod=Linear search  BeginIndexSearchUsingPreviousIndexResult=on  ExtrapMethod=Linear
  Prelookup1 : PreLookup  BreakpointsData=Aero.dC6_rud.beta  IndexSearchMethod=Linear search  BeginIndexSearchUsingPreviousIndexResult=on  ExtrapMethod=Linear
  Prelookup2 : PreLookup  BreakpointsData=Aero.dC6_rud.rud  IndexSearchMethod=Linear search  BeginIndexSearchUsingPreviousIndexResult=on  ExtrapMethod=Linear
  Product1 : Product  RndMeth=Zero
  Product2 : Product  RndMeth=Zero
  Switch : Switch
  dC6 : Outport
  wires:
  Constant2/1 -> Interpolation Using Prelookup/7
  Prelookup2/2 -> Interpolation Using Prelookup/6
  Prelookup2/1 -> Interpolation Using Prelookup/5
  Prelookup1/2 -> Interpolation Using Prelookup/4
  Prelookup1/1 -> Interpolation Using Prelookup/3
  Prelookup/2 -> Interpolation Using Prelookup/2
  Prelookup/1 -> Interpolation Using Prelookup/1
  Product1/1 -> Prelookup1/1
  rud/1 -> Abs/1, Switch/2
  Abs/1 -> Gain/1
  Gain/1 -> Prelookup2/1
  alpha/1 -> Prelookup/1
  beta/1 -> Product1/1
  Product2/1 -> dC6/1
  Constant/1 -> Switch/1
  Constant1/1 -> Switch/3
  Switch/1 -> Product1/2, Assignment to lateral/2
  Constant3/1 -> Assignment to lateral/1
  Assignment to lateral/1 -> Product2/2
  Interpolation Using Prelookup/1 -> Product2/1

== system gtm_design/GTM_T2/Aero/Control Surfaces/Spoilers/Gains1 ==
  dC6_in : Inport
  Product : Product  RndMeth=Zero
  gains : Constant  Value=gains
  dC6 : Outport
  wires:
  dC6_in/1 -> Product/1
  Product/1 -> dC6/1
  gains/1 -> Product/2

== system gtm_design/GTM_T2/Aero/Control Surfaces/Spoilers/Gains2 ==
  dC6_in : Inport
  Product : Product  RndMeth=Zero
  gains : Constant  Value=gains
  dC6 : Outport
  wires:
  gains/1 -> Product/2
  Product/1 -> dC6/1
  dC6_in/1 -> Product/1

== system gtm_design/GTM_T2/Aero/Control Surfaces/Spoilers/Gains3 ==
  dC6_in : Inport
  Product : Product  RndMeth=Zero
  gains : Constant  Value=gains
  dC6 : Outport
  wires:
  gains/1 -> Product/2
  Product/1 -> dC6/1
  dC6_in/1 -> Product/1

== system gtm_design/GTM_T2/Aero/Control Surfaces/Spoilers/Gains4 ==
  dC6_in : Inport
  Product : Product  RndMeth=Zero
  gains : Constant  Value=gains
  dC6 : Outport
  wires:
  dC6_in/1 -> Product/1
  Product/1 -> dC6/1
  gains/1 -> Product/2
